simulink model "t_type_three_phase_q1q4_switching"  (R2025b)
settings: Solver=ode23t  StartTime=0.0  StopTime=0.06  MaxStep=max_step_sw  RelTol=1e-3
PreLoadFcn:
  | demo_root=fileparts(fileparts(get_param(bdroot,'FileName'))); run(fullfile(demo_root,'parameters','closed_loop_demo_parameters.m')); clear demo_root;
undefined symbols (not defined in the file): dead_time_cl, m_index, Rd_sw, T_switch, Vdc_sw, w_grid_sw
libraries: ee_lib x29, nesl_utility x19, fl_lib x7, simulink x3
settings Model: Creator=bob  LastModifiedBy=bob

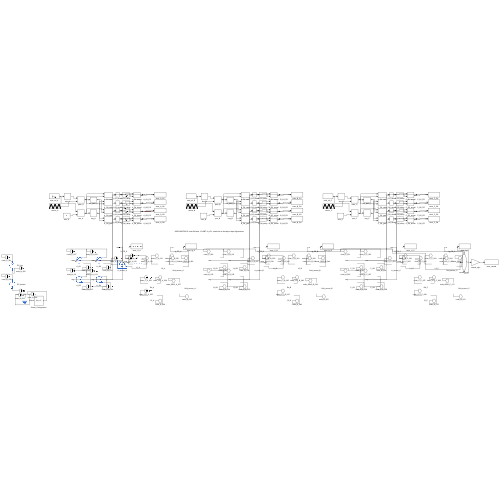
[thumbnail: Simulink's stored preview of the top-level diagram]
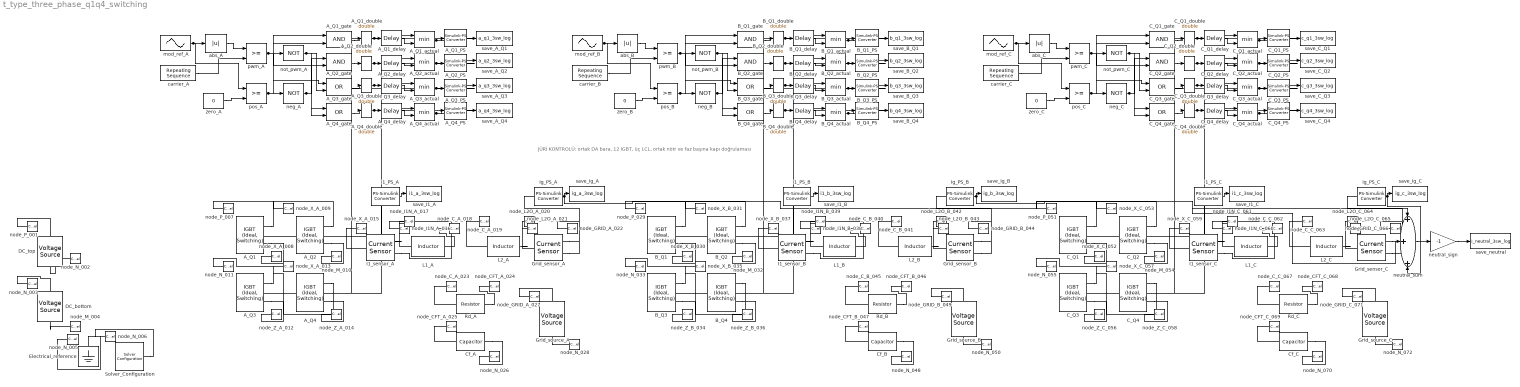
== system t_type_three_phase_q1q4_switching ==
  note: JÜRİ KONTROLÜ: ortak DA bara, 12 IGBT, üç LCL, ortak nötr ve faz başına kapı doğrulaması
  A_Q{1..4} (4 alike) : ee_lib/Semiconductors & Converters/IGBT (Ideal, Switching)  port_option=ee.enum.controlport.ps  Vf=Vf_sw V  Ron=Ron_sw Ohm  Goff=Goff_sw 1/Ohm  Vth=Vth_sw V  diode_param=ee.enum.semiconductors.protectionDiode.nodynamics  diode_Vf=0.8 V  diode_Ron=0.001 Ohm  diode_Goff=1e-5 1/Ohm  diode_C=50e-9 F  diode_iRM=-235 A  diode_iF=300 A  diode_idot=-50 A/us  diode_trr_param=ee.enum.converters.diodeReverseParam.trr_factor  diode_trr_factor=3  diode_trr=15 us  diode_Qrr=1500 s*uA  ice_specify=off  ice_priority=None  ice=0 A  ice_nominal_specify=off  ice_nominal_value=1  ice_nominal_unit=A  vce_specify=off  vce_priority=None  vce=0 V  vce_nominal_specify=off  vce_nominal_value=1  vce_nominal_unit=V  vge_specify=off  vge_priority=None  vge=0 V  vge_nominal_specify=off  vge_nominal_value=1  vge_nominal_unit=V  thermal_loss_option=ee.enum.converters.thermalLossOption.constantvalues  Von_data=[0, .1, .6, .8, 1, 1.3, 1.6, 2, 2.4; 0, .1, .7, 1, 1.2, 1.5, 1.9, 2.4, 2.8] V  Tj=[298.15, 398.15] K  Iout_data=[0, .1, 1, 5, 10, 20, 40, 70, 100] A  Eon_data=[0, .0024, .024, .12, .2, .48, 1.04, 2.16, 3.24; 0, .003, .03, .15, .25, .6, 1.3, 2.7, 4.05] * 1e-3 J  Eoff_data=[0, .0007, .0066, .033, .066, .17, .33, .83, 1.5; 0, .001, .01, .05, .1, .25, .5, 1.2, 2.2] * 1e-3 J  Eon_data_3D=[zeros(2, 9, 3)] J  Eoff_data_3D=[zeros(2, 9, 3)] J  Tj_loss=[298.15, 398.15] K  Iout_data_loss=[0, .1, 1, 5, 10, 20, 40, 70, 100] A  tabulateWithVce=false  Vce_loss=[0, 150, 300] V  Eon_scalar=22.86e-3 J  Eoff_scalar=17.14e-3 J  Voff=300 V  Iout_scalar=600 A  useCurrentFromPreviousCycle=false  useVoltageFromPreviousCycle=false  diodeModelType=ee.enum.converters.diodeModelType.pwl  diodeTableType=ee.enum.diode.tableType.IfMat  diode_ReverseIVType=ee.enum.diode.diodeReverseIV.constant  diode_IfMat=[.07, .12, .19, 1.75, 4.24, 7.32, 11.2; .16, .3, .72, 2.14, 4.02, 6.35, 9.12] A  diode_VfMat=[.9, 1.15, 1.25, 1.5, 1.75, 2.17, 2.6, 2.85; .58, .68, .75, 1.1, 1.38, 1.77, 2.27, 2.7] V  diode_TjVec=[25, 125] degC  diode_VfVec=[.5, .7, .9, 1.3, 1.7, 2.1, 2.5] V  diode_IfVec=[.1, .2, .5, 1, 2, 4, 7, 10] A  diode_IrMat=[1e-06, 2e-06, 5e-06, 1e-05, 2.5e-05, 5e-05, .0001; 2e-06, 5e-06, 1e-05, 4e-05, 8e-05, .0002, .0005] A  diode_VrMat=[10, 100, 200, 250, 300, 325, 350; 10, 70, 160, 220, 270, 300, 320] V  diode_VrVec=[10, 20, 40, 50, 70, 80, 100] V  diode_IrVec=[1e-06, 2e-06, 5e-06, 1e-05, 2e-05, 5e-05, .0001] A  diode_Vr=-600 V  diode_Ls=150 nH  diode_Erec=0.03 J  diode_rec_loss_model=ee.enum.diode.reverseRecoveryModel.fixed  diode_ErecVal=0 J  diode_scaleWithIandV=true  diode_ErecMat=zeros(2, 3) J  diode_TjrecVec=[298.15, 398.15] K  diode_IfrecVec=[.1, 1, 10] A  diode_IrecVal=10 A  diode_VrecVal=10 V  diode_tFilter=1 / 1000 / 100 s  separateThermalPortForDiode=false  thermal_network_parameterization=ee.enum.thermalNetworkTopology.external  Rth=[.08, .5] K/W  Rth_Cauer=[.08, .1, .5] K/W  Rth_Foster=[.08, .14, .22, .16] K/W  thermal_mass_parameterization=ee.enum.thermalNetwork.timeconstant  thermal_mass=[.01, .5] J/K  thermal_mass_Cauer=[.01, .1, .5] J/K  thermal_mass_Foster=[.001, .005, .05, .5] J/K  thermal_time_constant=[.001, .2] s  thermal_time_constant_Cauer=[.001, .1, .2] s  thermal_time_constant_Foster=[7e-05, .0007, .01, .08] s  thermal_mass_initial_temperatures=[25, 25] degC  thermal_mass_initial_temperatures_Cauer=[25, 25, 25] degC  junction_thermal_mass=0.01 J/K  Tvec_initial_Foster=[25, 25, 25, 25] degC  RthDiode=[.03, .2] K/W  RthCauerDiode=[.03, .1, .2] K/W  RthFosterDiode=[.03, .2] K/W  thermalMassDiode=[3, 25] J/K  thermalMassCauerDiode=[3, 10, 25] J/K  thermalMassFosterDiode=[33, 50] J/K  thermalTauDiode=[.1, 5] s  thermalTauCauerDiode=[.1, 1, 5] s  thermalTauFosterDiode=[1, 10] s  thermalMassInitTempDiode=[25, 25] degC  thermalMassInitTempCauerDiode=[25, 25, 25] degC  junctionthermalMassDiode=0.1 J/K  TVecInitialFosterDiode=[25, 25, 25, 25] degC  no_thermal_network=0  IGBT_junction_temperature_specify=off  IGBT_junction_temperature_priority=None  IGBT_junction_temperature=25 degC  IGBT_junction_temperature_nominal_specify=off  IGBT_junction_temperature_nominal_value=1  IGBT_junction_temperature_nominal_unit=degC  diode_junction_temperature_specify=off  diode_junction_temperature_priority=None  diode_junction_temperature=25 degC  diode_junction_temperature_nominal_specify=off  diode_junction_temperature_nominal_value=1  diode_junction_temperature_nominal_unit=degC  Qj_specify=off  Qj_priority=None  Qj=0 W  Qj_nominal_specify=off  Qj_nominal_value=1  Qj_nominal_unit=W  accumulatedSwitchingLosses_specify=off  accumulatedSwitchingLosses_priority=None  accumulatedSwitchingLosses=0 J
  A_Q1_PS : nesl_utility/Simulink-PS Converter  PhysicalDomain=network_engine_domain  SubClassName=ps_input  LeftPortType=input  RightPortType=output  PseudoPeriodic=off  Frequencies=[]  NoiseDistribution=none  NoiseParameters=[]  Unit=V  AffineConversion=off  FilteringAndDerivatives=zero  SimscapeFilterOrder=1  InputFilterTimeConstant=0.001  UdotUserProvided=0
  A_Q1_actual : MinMax  Inputs=2
  A_Q1_delay : TransportDelay  DelayTime=dead_time_cl
  A_Q1_double : DataTypeConversion  OutDataTypeStr=double  SaturateOnIntegerOverflow=off  RndMeth=Floor
  A_Q1_gate : Logic  AllPortsSameDT=off  OutDataTypeStr=boolean
  A_Q2_PS : nesl_utility/Simulink-PS Converter  PhysicalDomain=network_engine_domain  SubClassName=ps_input  LeftPortType=input  RightPortType=output  PseudoPeriodic=off  Frequencies=[]  NoiseDistribution=none  NoiseParameters=[]  Unit=V  AffineConversion=off  FilteringAndDerivatives=zero  SimscapeFilterOrder=1  InputFilterTimeConstant=0.001  UdotUserProvided=0
  A_Q2_actual : MinMax  Inputs=2
  A_Q2_delay : TransportDelay  DelayTime=dead_time_cl
  A_Q2_double : DataTypeConversion  OutDataTypeStr=double  SaturateOnIntegerOverflow=off  RndMeth=Floor
  A_Q2_gate : Logic  AllPortsSameDT=off  OutDataTypeStr=boolean
  A_Q3_PS : nesl_utility/Simulink-PS Converter  PhysicalDomain=network_engine_domain  SubClassName=ps_input  LeftPortType=input  RightPortType=output  PseudoPeriodic=off  Frequencies=[]  NoiseDistribution=none  NoiseParameters=[]  Unit=V  AffineConversion=off  FilteringAndDerivatives=zero  SimscapeFilterOrder=1  InputFilterTimeConstant=0.001  UdotUserProvided=0
  A_Q3_actual : MinMax  Inputs=2
  A_Q3_delay : TransportDelay  DelayTime=dead_time_cl
  A_Q3_double : DataTypeConversion  OutDataTypeStr=double  SaturateOnIntegerOverflow=off  RndMeth=Floor
  A_Q3_gate : Logic  Operator=OR  AllPortsSameDT=off  OutDataTypeStr=boolean
  A_Q4_PS : nesl_utility/Simulink-PS Converter  PhysicalDomain=network_engine_domain  SubClassName=ps_input  LeftPortType=input  RightPortType=output  PseudoPeriodic=off  Frequencies=[]  NoiseDistribution=none  NoiseParameters=[]  Unit=V  AffineConversion=off  FilteringAndDerivatives=zero  SimscapeFilterOrder=1  InputFilterTimeConstant=0.001  UdotUserProvided=0
  A_Q4_actual : MinMax  Inputs=2
  A_Q4_delay : TransportDelay  DelayTime=dead_time_cl
  A_Q4_double : DataTypeConversion  OutDataTypeStr=double  SaturateOnIntegerOverflow=off  RndMeth=Floor
  A_Q4_gate : Logic  Operator=OR  AllPortsSameDT=off  OutDataTypeStr=boolean
  B_Q{1..4} (4 alike) : ee_lib/Semiconductors & Converters/IGBT (Ideal, Switching)  port_option=ee.enum.controlport.ps  Vf=Vf_sw V  Ron=Ron_sw Ohm  Goff=Goff_sw 1/Ohm  Vth=Vth_sw V  diode_param=ee.enum.semiconductors.protectionDiode.nodynamics  diode_Vf=0.8 V  diode_Ron=0.001 Ohm  diode_Goff=1e-5 1/Ohm  diode_C=50e-9 F  diode_iRM=-235 A  diode_iF=300 A  diode_idot=-50 A/us  diode_trr_param=ee.enum.converters.diodeReverseParam.trr_factor  diode_trr_factor=3  diode_trr=15 us  diode_Qrr=1500 s*uA  ice_specify=off  ice_priority=None  ice=0 A  ice_nominal_specify=off  ice_nominal_value=1  ice_nominal_unit=A  vce_specify=off  vce_priority=None  vce=0 V  vce_nominal_specify=off  vce_nominal_value=1  vce_nominal_unit=V  vge_specify=off  vge_priority=None  vge=0 V  vge_nominal_specify=off  vge_nominal_value=1  vge_nominal_unit=V  thermal_loss_option=ee.enum.converters.thermalLossOption.constantvalues  Von_data=[0, .1, .6, .8, 1, 1.3, 1.6, 2, 2.4; 0, .1, .7, 1, 1.2, 1.5, 1.9, 2.4, 2.8] V  Tj=[298.15, 398.15] K  Iout_data=[0, .1, 1, 5, 10, 20, 40, 70, 100] A  Eon_data=[0, .0024, .024, .12, .2, .48, 1.04, 2.16, 3.24; 0, .003, .03, .15, .25, .6, 1.3, 2.7, 4.05] * 1e-3 J  Eoff_data=[0, .0007, .0066, .033, .066, .17, .33, .83, 1.5; 0, .001, .01, .05, .1, .25, .5, 1.2, 2.2] * 1e-3 J  Eon_data_3D=[zeros(2, 9, 3)] J  Eoff_data_3D=[zeros(2, 9, 3)] J  Tj_loss=[298.15, 398.15] K  Iout_data_loss=[0, .1, 1, 5, 10, 20, 40, 70, 100] A  tabulateWithVce=false  Vce_loss=[0, 150, 300] V  Eon_scalar=22.86e-3 J  Eoff_scalar=17.14e-3 J  Voff=300 V  Iout_scalar=600 A  useCurrentFromPreviousCycle=false  useVoltageFromPreviousCycle=false  diodeModelType=ee.enum.converters.diodeModelType.pwl  diodeTableType=ee.enum.diode.tableType.IfMat  diode_ReverseIVType=ee.enum.diode.diodeReverseIV.constant  diode_IfMat=[.07, .12, .19, 1.75, 4.24, 7.32, 11.2; .16, .3, .72, 2.14, 4.02, 6.35, 9.12] A  diode_VfMat=[.9, 1.15, 1.25, 1.5, 1.75, 2.17, 2.6, 2.85; .58, .68, .75, 1.1, 1.38, 1.77, 2.27, 2.7] V  diode_TjVec=[25, 125] degC  diode_VfVec=[.5, .7, .9, 1.3, 1.7, 2.1, 2.5] V  diode_IfVec=[.1, .2, .5, 1, 2, 4, 7, 10] A  diode_IrMat=[1e-06, 2e-06, 5e-06, 1e-05, 2.5e-05, 5e-05, .0001; 2e-06, 5e-06, 1e-05, 4e-05, 8e-05, .0002, .0005] A  diode_VrMat=[10, 100, 200, 250, 300, 325, 350; 10, 70, 160, 220, 270, 300, 320] V  diode_VrVec=[10, 20, 40, 50, 70, 80, 100] V  diode_IrVec=[1e-06, 2e-06, 5e-06, 1e-05, 2e-05, 5e-05, .0001] A  diode_Vr=-600 V  diode_Ls=150 nH  diode_Erec=0.03 J  diode_rec_loss_model=ee.enum.diode.reverseRecoveryModel.fixed  diode_ErecVal=0 J  diode_scaleWithIandV=true  diode_ErecMat=zeros(2, 3) J  diode_TjrecVec=[298.15, 398.15] K  diode_IfrecVec=[.1, 1, 10] A  diode_IrecVal=10 A  diode_VrecVal=10 V  diode_tFilter=1 / 1000 / 100 s  separateThermalPortForDiode=false  thermal_network_parameterization=ee.enum.thermalNetworkTopology.external  Rth=[.08, .5] K/W  Rth_Cauer=[.08, .1, .5] K/W  Rth_Foster=[.08, .14, .22, .16] K/W  thermal_mass_parameterization=ee.enum.thermalNetwork.timeconstant  thermal_mass=[.01, .5] J/K  thermal_mass_Cauer=[.01, .1, .5] J/K  thermal_mass_Foster=[.001, .005, .05, .5] J/K  thermal_time_constant=[.001, .2] s  thermal_time_constant_Cauer=[.001, .1, .2] s  thermal_time_constant_Foster=[7e-05, .0007, .01, .08] s  thermal_mass_initial_temperatures=[25, 25] degC  thermal_mass_initial_temperatures_Cauer=[25, 25, 25] degC  junction_thermal_mass=0.01 J/K  Tvec_initial_Foster=[25, 25, 25, 25] degC  RthDiode=[.03, .2] K/W  RthCauerDiode=[.03, .1, .2] K/W  RthFosterDiode=[.03, .2] K/W  thermalMassDiode=[3, 25] J/K  thermalMassCauerDiode=[3, 10, 25] J/K  thermalMassFosterDiode=[33, 50] J/K  thermalTauDiode=[.1, 5] s  thermalTauCauerDiode=[.1, 1, 5] s  thermalTauFosterDiode=[1, 10] s  thermalMassInitTempDiode=[25, 25] degC  thermalMassInitTempCauerDiode=[25, 25, 25] degC  junctionthermalMassDiode=0.1 J/K  TVecInitialFosterDiode=[25, 25, 25, 25] degC  no_thermal_network=0  IGBT_junction_temperature_specify=off  IGBT_junction_temperature_priority=None  IGBT_junction_temperature=25 degC  IGBT_junction_temperature_nominal_specify=off  IGBT_junction_temperature_nominal_value=1  IGBT_junction_temperature_nominal_unit=degC  diode_junction_temperature_specify=off  diode_junction_temperature_priority=None  diode_junction_temperature=25 degC  diode_junction_temperature_nominal_specify=off  diode_junction_temperature_nominal_value=1  diode_junction_temperature_nominal_unit=degC  Qj_specify=off  Qj_priority=None  Qj=0 W  Qj_nominal_specify=off  Qj_nominal_value=1  Qj_nominal_unit=W  accumulatedSwitchingLosses_specify=off  accumulatedSwitchingLosses_priority=None  accumulatedSwitchingLosses=0 J
  B_Q1_PS : nesl_utility/Simulink-PS Converter  PhysicalDomain=network_engine_domain  SubClassName=ps_input  LeftPortType=input  RightPortType=output  PseudoPeriodic=off  Frequencies=[]  NoiseDistribution=none  NoiseParameters=[]  Unit=V  AffineConversion=off  FilteringAndDerivatives=zero  SimscapeFilterOrder=1  InputFilterTimeConstant=0.001  UdotUserProvided=0
  B_Q1_actual : MinMax  Inputs=2
  B_Q1_delay : TransportDelay  DelayTime=dead_time_cl
  B_Q1_double : DataTypeConversion  OutDataTypeStr=double  SaturateOnIntegerOverflow=off  RndMeth=Floor
  B_Q1_gate : Logic  AllPortsSameDT=off  OutDataTypeStr=boolean
  B_Q2_PS : nesl_utility/Simulink-PS Converter  PhysicalDomain=network_engine_domain  SubClassName=ps_input  LeftPortType=input  RightPortType=output  PseudoPeriodic=off  Frequencies=[]  NoiseDistribution=none  NoiseParameters=[]  Unit=V  AffineConversion=off  FilteringAndDerivatives=zero  SimscapeFilterOrder=1  InputFilterTimeConstant=0.001  UdotUserProvided=0
  B_Q2_actual : MinMax  Inputs=2
  B_Q2_delay : TransportDelay  DelayTime=dead_time_cl
  B_Q2_double : DataTypeConversion  OutDataTypeStr=double  SaturateOnIntegerOverflow=off  RndMeth=Floor
  B_Q2_gate : Logic  AllPortsSameDT=off  OutDataTypeStr=boolean
  B_Q3_PS : nesl_utility/Simulink-PS Converter  PhysicalDomain=network_engine_domain  SubClassName=ps_input  LeftPortType=input  RightPortType=output  PseudoPeriodic=off  Frequencies=[]  NoiseDistribution=none  NoiseParameters=[]  Unit=V  AffineConversion=off  FilteringAndDerivatives=zero  SimscapeFilterOrder=1  InputFilterTimeConstant=0.001  UdotUserProvided=0
  B_Q3_actual : MinMax  Inputs=2
  B_Q3_delay : TransportDelay  DelayTime=dead_time_cl
  B_Q3_double : DataTypeConversion  OutDataTypeStr=double  SaturateOnIntegerOverflow=off  RndMeth=Floor
  B_Q3_gate : Logic  Operator=OR  AllPortsSameDT=off  OutDataTypeStr=boolean
  B_Q4_PS : nesl_utility/Simulink-PS Converter  PhysicalDomain=network_engine_domain  SubClassName=ps_input  LeftPortType=input  RightPortType=output  PseudoPeriodic=off  Frequencies=[]  NoiseDistribution=none  NoiseParameters=[]  Unit=V  AffineConversion=off  FilteringAndDerivatives=zero  SimscapeFilterOrder=1  InputFilterTimeConstant=0.001  UdotUserProvided=0
  B_Q4_actual : MinMax  Inputs=2
  B_Q4_delay : TransportDelay  DelayTime=dead_time_cl
  B_Q4_double : DataTypeConversion  OutDataTypeStr=double  SaturateOnIntegerOverflow=off  RndMeth=Floor
  B_Q4_gate : Logic  Operator=OR  AllPortsSameDT=off  OutDataTypeStr=boolean
  C_Q{1..4} (4 alike) : ee_lib/Semiconductors & Converters/IGBT (Ideal, Switching)  port_option=ee.enum.controlport.ps  Vf=Vf_sw V  Ron=Ron_sw Ohm  Goff=Goff_sw 1/Ohm  Vth=Vth_sw V  diode_param=ee.enum.semiconductors.protectionDiode.nodynamics  diode_Vf=0.8 V  diode_Ron=0.001 Ohm  diode_Goff=1e-5 1/Ohm  diode_C=50e-9 F  diode_iRM=-235 A  diode_iF=300 A  diode_idot=-50 A/us  diode_trr_param=ee.enum.converters.diodeReverseParam.trr_factor  diode_trr_factor=3  diode_trr=15 us  diode_Qrr=1500 s*uA  ice_specify=off  ice_priority=None  ice=0 A  ice_nominal_specify=off  ice_nominal_value=1  ice_nominal_unit=A  vce_specify=off  vce_priority=None  vce=0 V  vce_nominal_specify=off  vce_nominal_value=1  vce_nominal_unit=V  vge_specify=off  vge_priority=None  vge=0 V  vge_nominal_specify=off  vge_nominal_value=1  vge_nominal_unit=V  thermal_loss_option=ee.enum.converters.thermalLossOption.constantvalues  Von_data=[0, .1, .6, .8, 1, 1.3, 1.6, 2, 2.4; 0, .1, .7, 1, 1.2, 1.5, 1.9, 2.4, 2.8] V  Tj=[298.15, 398.15] K  Iout_data=[0, .1, 1, 5, 10, 20, 40, 70, 100] A  Eon_data=[0, .0024, .024, .12, .2, .48, 1.04, 2.16, 3.24; 0, .003, .03, .15, .25, .6, 1.3, 2.7, 4.05] * 1e-3 J  Eoff_data=[0, .0007, .0066, .033, .066, .17, .33, .83, 1.5; 0, .001, .01, .05, .1, .25, .5, 1.2, 2.2] * 1e-3 J  Eon_data_3D=[zeros(2, 9, 3)] J  Eoff_data_3D=[zeros(2, 9, 3)] J  Tj_loss=[298.15, 398.15] K  Iout_data_loss=[0, .1, 1, 5, 10, 20, 40, 70, 100] A  tabulateWithVce=false  Vce_loss=[0, 150, 300] V  Eon_scalar=22.86e-3 J  Eoff_scalar=17.14e-3 J  Voff=300 V  Iout_scalar=600 A  useCurrentFromPreviousCycle=false  useVoltageFromPreviousCycle=false  diodeModelType=ee.enum.converters.diodeModelType.pwl  diodeTableType=ee.enum.diode.tableType.IfMat  diode_ReverseIVType=ee.enum.diode.diodeReverseIV.constant  diode_IfMat=[.07, .12, .19, 1.75, 4.24, 7.32, 11.2; .16, .3, .72, 2.14, 4.02, 6.35, 9.12] A  diode_VfMat=[.9, 1.15, 1.25, 1.5, 1.75, 2.17, 2.6, 2.85; .58, .68, .75, 1.1, 1.38, 1.77, 2.27, 2.7] V  diode_TjVec=[25, 125] degC  diode_VfVec=[.5, .7, .9, 1.3, 1.7, 2.1, 2.5] V  diode_IfVec=[.1, .2, .5, 1, 2, 4, 7, 10] A  diode_IrMat=[1e-06, 2e-06, 5e-06, 1e-05, 2.5e-05, 5e-05, .0001; 2e-06, 5e-06, 1e-05, 4e-05, 8e-05, .0002, .0005] A  diode_VrMat=[10, 100, 200, 250, 300, 325, 350; 10, 70, 160, 220, 270, 300, 320] V  diode_VrVec=[10, 20, 40, 50, 70, 80, 100] V  diode_IrVec=[1e-06, 2e-06, 5e-06, 1e-05, 2e-05, 5e-05, .0001] A  diode_Vr=-600 V  diode_Ls=150 nH  diode_Erec=0.03 J  diode_rec_loss_model=ee.enum.diode.reverseRecoveryModel.fixed  diode_ErecVal=0 J  diode_scaleWithIandV=true  diode_ErecMat=zeros(2, 3) J  diode_TjrecVec=[298.15, 398.15] K  diode_IfrecVec=[.1, 1, 10] A  diode_IrecVal=10 A  diode_VrecVal=10 V  diode_tFilter=1 / 1000 / 100 s  separateThermalPortForDiode=false  thermal_network_parameterization=ee.enum.thermalNetworkTopology.external  Rth=[.08, .5] K/W  Rth_Cauer=[.08, .1, .5] K/W  Rth_Foster=[.08, .14, .22, .16] K/W  thermal_mass_parameterization=ee.enum.thermalNetwork.timeconstant  thermal_mass=[.01, .5] J/K  thermal_mass_Cauer=[.01, .1, .5] J/K  thermal_mass_Foster=[.001, .005, .05, .5] J/K  thermal_time_constant=[.001, .2] s  thermal_time_constant_Cauer=[.001, .1, .2] s  thermal_time_constant_Foster=[7e-05, .0007, .01, .08] s  thermal_mass_initial_temperatures=[25, 25] degC  thermal_mass_initial_temperatures_Cauer=[25, 25, 25] degC  junction_thermal_mass=0.01 J/K  Tvec_initial_Foster=[25, 25, 25, 25] degC  RthDiode=[.03, .2] K/W  RthCauerDiode=[.03, .1, .2] K/W  RthFosterDiode=[.03, .2] K/W  thermalMassDiode=[3, 25] J/K  thermalMassCauerDiode=[3, 10, 25] J/K  thermalMassFosterDiode=[33, 50] J/K  thermalTauDiode=[.1, 5] s  thermalTauCauerDiode=[.1, 1, 5] s  thermalTauFosterDiode=[1, 10] s  thermalMassInitTempDiode=[25, 25] degC  thermalMassInitTempCauerDiode=[25, 25, 25] degC  junctionthermalMassDiode=0.1 J/K  TVecInitialFosterDiode=[25, 25, 25, 25] degC  no_thermal_network=0  IGBT_junction_temperature_specify=off  IGBT_junction_temperature_priority=None  IGBT_junction_temperature=25 degC  IGBT_junction_temperature_nominal_specify=off  IGBT_junction_temperature_nominal_value=1  IGBT_junction_temperature_nominal_unit=degC  diode_junction_temperature_specify=off  diode_junction_temperature_priority=None  diode_junction_temperature=25 degC  diode_junction_temperature_nominal_specify=off  diode_junction_temperature_nominal_value=1  diode_junction_temperature_nominal_unit=degC  Qj_specify=off  Qj_priority=None  Qj=0 W  Qj_nominal_specify=off  Qj_nominal_value=1  Qj_nominal_unit=W  accumulatedSwitchingLosses_specify=off  accumulatedSwitchingLosses_priority=None  accumulatedSwitchingLosses=0 J
  C_Q1_PS : nesl_utility/Simulink-PS Converter  PhysicalDomain=network_engine_domain  SubClassName=ps_input  LeftPortType=input  RightPortType=output  PseudoPeriodic=off  Frequencies=[]  NoiseDistribution=none  NoiseParameters=[]  Unit=V  AffineConversion=off  FilteringAndDerivatives=zero  SimscapeFilterOrder=1  InputFilterTimeConstant=0.001  UdotUserProvided=0
  C_Q1_actual : MinMax  Inputs=2
  C_Q1_delay : TransportDelay  DelayTime=dead_time_cl
  C_Q1_double : DataTypeConversion  OutDataTypeStr=double  SaturateOnIntegerOverflow=off  RndMeth=Floor
  C_Q1_gate : Logic  AllPortsSameDT=off  OutDataTypeStr=boolean
  C_Q2_PS : nesl_utility/Simulink-PS Converter  PhysicalDomain=network_engine_domain  SubClassName=ps_input  LeftPortType=input  RightPortType=output  PseudoPeriodic=off  Frequencies=[]  NoiseDistribution=none  NoiseParameters=[]  Unit=V  AffineConversion=off  FilteringAndDerivatives=zero  SimscapeFilterOrder=1  InputFilterTimeConstant=0.001  UdotUserProvided=0
  C_Q2_actual : MinMax  Inputs=2
  C_Q2_delay : TransportDelay  DelayTime=dead_time_cl
  C_Q2_double : DataTypeConversion  OutDataTypeStr=double  SaturateOnIntegerOverflow=off  RndMeth=Floor
  C_Q2_gate : Logic  AllPortsSameDT=off  OutDataTypeStr=boolean
  C_Q3_PS : nesl_utility/Simulink-PS Converter  PhysicalDomain=network_engine_domain  SubClassName=ps_input  LeftPortType=input  RightPortType=output  PseudoPeriodic=off  Frequencies=[]  NoiseDistribution=none  NoiseParameters=[]  Unit=V  AffineConversion=off  FilteringAndDerivatives=zero  SimscapeFilterOrder=1  InputFilterTimeConstant=0.001  UdotUserProvided=0
  C_Q3_actual : MinMax  Inputs=2
  C_Q3_delay : TransportDelay  DelayTime=dead_time_cl
  C_Q3_double : DataTypeConversion  OutDataTypeStr=double  SaturateOnIntegerOverflow=off  RndMeth=Floor
  C_Q3_gate : Logic  Operator=OR  AllPortsSameDT=off  OutDataTypeStr=boolean
  C_Q4_PS : nesl_utility/Simulink-PS Converter  PhysicalDomain=network_engine_domain  SubClassName=ps_input  LeftPortType=input  RightPortType=output  PseudoPeriodic=off  Frequencies=[]  NoiseDistribution=none  NoiseParameters=[]  Unit=V  AffineConversion=off  FilteringAndDerivatives=zero  SimscapeFilterOrder=1  InputFilterTimeConstant=0.001  UdotUserProvided=0
  C_Q4_actual : MinMax  Inputs=2
  C_Q4_delay : TransportDelay  DelayTime=dead_time_cl
  C_Q4_double : DataTypeConversion  OutDataTypeStr=double  SaturateOnIntegerOverflow=off  RndMeth=Floor
  C_Q4_gate : Logic  Operator=OR  AllPortsSameDT=off  OutDataTypeStr=boolean
  Cf_A : ee_lib/Passive/Capacitor  cap_option=ee.enum.passive.capacitor.capOption.const  c=Cf_sw F  Cvec=[1e-05, 1e-06] F  Vvec=[0, 10] V  CV_table_symmetry=ee.enum.passive.capacitor.tableSymmetry.yes  f_vec=[1, 10] kHz  DFext_vec=[.8, 1.2]  enable_C_tol=ee.enum.toleranceApplication.none  averaging_period=0 s  C_tol=5  tol_distribution=ee.enum.toleranceDistribution.uniform  nSigma=4  r=0 Ohm  g=0 1/Ohm  enable_operating_limits=ee.enum.enable.no  operating_limit_action=ee.enum.passive.reportOpLim.warn  max_working_voltage_range=[-25, 25] V  power_rating=1 W  maxTemperature=85 degC  thermalEnable=false  thermalMass=1 J/K  i_specify=off  i_priority=None  i=0 A  i_nominal_specify=off  i_nominal_value=1  i_nominal_unit=A  v_specify=off  v_priority=None  v=0 V  v_nominal_specify=off  v_nominal_value=1  v_nominal_unit=V  vc_specify=off  vc_priority=High  vc=0 V  vc_nominal_specify=off  vc_nominal_value=1  vc_nominal_unit=V  T_specify=off  T_priority=None  T=298.15 K  T_nominal_specify=off  T_nominal_value=1  T_nominal_unit=K
  Cf_B : ee_lib/Passive/Capacitor  cap_option=ee.enum.passive.capacitor.capOption.const  c=Cf_sw F  Cvec=[1e-05, 1e-06] F  Vvec=[0, 10] V  CV_table_symmetry=ee.enum.passive.capacitor.tableSymmetry.yes  f_vec=[1, 10] kHz  DFext_vec=[.8, 1.2]  enable_C_tol=ee.enum.toleranceApplication.none  averaging_period=0 s  C_tol=5  tol_distribution=ee.enum.toleranceDistribution.uniform  nSigma=4  r=0 Ohm  g=0 1/Ohm  enable_operating_limits=ee.enum.enable.no  operating_limit_action=ee.enum.passive.reportOpLim.warn  max_working_voltage_range=[-25, 25] V  power_rating=1 W  maxTemperature=85 degC  thermalEnable=false  thermalMass=1 J/K  i_specify=off  i_priority=None  i=0 A  i_nominal_specify=off  i_nominal_value=1  i_nominal_unit=A  v_specify=off  v_priority=None  v=0 V  v_nominal_specify=off  v_nominal_value=1  v_nominal_unit=V  vc_specify=off  vc_priority=High  vc=0 V  vc_nominal_specify=off  vc_nominal_value=1  vc_nominal_unit=V  T_specify=off  T_priority=None  T=298.15 K  T_nominal_specify=off  T_nominal_value=1  T_nominal_unit=K
  Cf_C : ee_lib/Passive/Capacitor  cap_option=ee.enum.passive.capacitor.capOption.const  c=Cf_sw F  Cvec=[1e-05, 1e-06] F  Vvec=[0, 10] V  CV_table_symmetry=ee.enum.passive.capacitor.tableSymmetry.yes  f_vec=[1, 10] kHz  DFext_vec=[.8, 1.2]  enable_C_tol=ee.enum.toleranceApplication.none  averaging_period=0 s  C_tol=5  tol_distribution=ee.enum.toleranceDistribution.uniform  nSigma=4  r=0 Ohm  g=0 1/Ohm  enable_operating_limits=ee.enum.enable.no  operating_limit_action=ee.enum.passive.reportOpLim.warn  max_working_voltage_range=[-25, 25] V  power_rating=1 W  maxTemperature=85 degC  thermalEnable=false  thermalMass=1 J/K  i_specify=off  i_priority=None  i=0 A  i_nominal_specify=off  i_nominal_value=1  i_nominal_unit=A  v_specify=off  v_priority=None  v=0 V  v_nominal_specify=off  v_nominal_value=1  v_nominal_unit=V  vc_specify=off  vc_priority=High  vc=0 V  vc_nominal_specify=off  vc_nominal_value=1  vc_nominal_unit=V  T_specify=off  T_priority=None  T=298.15 K  T_nominal_specify=off  T_nominal_value=1  T_nominal_unit=K
  DC_bottom : ee_lib/Sources/Voltage Source  dc_voltage=Vdc_sw/2 V  ac_voltage=0 V  ac_shift=0 rad  ac_frequency=60 Hz  noise_mode=ee.enum.sources.noise.Disabled  PSD=0 V^2/Hz  sample_time=1e-3 s  repeatability=ee.enum.sources.repeatability.NotRepeatable  user_seed=0  auto_seed=3890346746  i_specify=off  i_priority=None  i=0 A  i_nominal_specify=off  i_nominal_value=1  i_nominal_unit=A  v_specify=off  v_priority=None  v=0 V  v_nominal_specify=off  v_nominal_value=1  v_nominal_unit=V
  DC_top : ee_lib/Sources/Voltage Source  dc_voltage=Vdc_sw/2 V  ac_voltage=0 V  ac_shift=0 rad  ac_frequency=60 Hz  noise_mode=ee.enum.sources.noise.Disabled  PSD=0 V^2/Hz  sample_time=1e-3 s  repeatability=ee.enum.sources.repeatability.NotRepeatable  user_seed=0  auto_seed=3499211588  i_specify=off  i_priority=None  i=0 A  i_nominal_specify=off  i_nominal_value=1  i_nominal_unit=A  v_specify=off  v_priority=None  v=0 V  v_nominal_specify=off  v_nominal_value=1  v_nominal_unit=V
  Electrical_reference : fl_lib/Electrical/Electrical Elements/Electrical Reference
  Grid_sensor_A : fl_lib/Electrical/Electrical Sensors/Current Sensor
  Grid_sensor_B : fl_lib/Electrical/Electrical Sensors/Current Sensor
  Grid_sensor_C : fl_lib/Electrical/Electrical Sensors/Current Sensor
  Grid_source_A : ee_lib/Sources/Voltage Source  dc_voltage=0 V  ac_voltage=V_grid_pk_sw V  ac_shift=0 rad  ac_frequency=f_grid_sw Hz  noise_mode=ee.enum.sources.noise.Disabled  PSD=0 V^2/Hz  sample_time=1e-3 s  repeatability=ee.enum.sources.repeatability.NotRepeatable  user_seed=0  auto_seed=3922919431  i_specify=off  i_priority=None  i=0 A  i_nominal_specify=off  i_nominal_value=1  i_nominal_unit=A  v_specify=off  v_priority=None  v=0 V  v_nominal_specify=off  v_nominal_value=1  v_nominal_unit=V
  Grid_source_B : ee_lib/Sources/Voltage Source  dc_voltage=0 V  ac_voltage=V_grid_pk_sw V  ac_shift=-2.0943951023931953 rad  ac_frequency=f_grid_sw Hz  noise_mode=ee.enum.sources.noise.Disabled  PSD=0 V^2/Hz  sample_time=1e-3 s  repeatability=ee.enum.sources.repeatability.NotRepeatable  user_seed=0  auto_seed=418932850  i_specify=off  i_priority=None  i=0 A  i_nominal_specify=off  i_nominal_value=1  i_nominal_unit=A  v_specify=off  v_priority=None  v=0 V  v_nominal_specify=off  v_nominal_value=1  v_nominal_unit=V
  Grid_source_C : ee_lib/Sources/Voltage Source  dc_voltage=0 V  ac_voltage=V_grid_pk_sw V  ac_shift=2.0943951023931953 rad  ac_frequency=f_grid_sw Hz  noise_mode=ee.enum.sources.noise.Disabled  PSD=0 V^2/Hz  sample_time=1e-3 s  repeatability=ee.enum.sources.repeatability.NotRepeatable  user_seed=0  auto_seed=2348838240  i_specify=off  i_priority=None  i=0 A  i_nominal_specify=off  i_nominal_value=1  i_nominal_unit=A  v_specify=off  v_priority=None  v=0 V  v_nominal_specify=off  v_nominal_value=1  v_nominal_unit=V
  I1_PS_A : nesl_utility/PS-Simulink Converter  PhysicalDomain=network_engine_domain  SubClassName=ps_output  LeftPortType=input  RightPortType=output  PseudoPeriodic=off  Frequencies=[]  VectorFormat=inherit  Unit=A  AffineConversion=off
  I1_PS_B : nesl_utility/PS-Simulink Converter  PhysicalDomain=network_engine_domain  SubClassName=ps_output  LeftPortType=input  RightPortType=output  PseudoPeriodic=off  Frequencies=[]  VectorFormat=inherit  Unit=A  AffineConversion=off
  I1_PS_C : nesl_utility/PS-Simulink Converter  PhysicalDomain=network_engine_domain  SubClassName=ps_output  LeftPortType=input  RightPortType=output  PseudoPeriodic=off  Frequencies=[]  VectorFormat=inherit  Unit=A  AffineConversion=off
  I1_sensor_A : fl_lib/Electrical/Electrical Sensors/Current Sensor
  I1_sensor_B : fl_lib/Electrical/Electrical Sensors/Current Sensor
  I1_sensor_C : fl_lib/Electrical/Electrical Sensors/Current Sensor
  Ig_PS_A : nesl_utility/PS-Simulink Converter  PhysicalDomain=network_engine_domain  SubClassName=ps_output  LeftPortType=input  RightPortType=output  PseudoPeriodic=off  Frequencies=[]  VectorFormat=inherit  Unit=A  AffineConversion=off
  Ig_PS_B : nesl_utility/PS-Simulink Converter  PhysicalDomain=network_engine_domain  SubClassName=ps_output  LeftPortType=input  RightPortType=output  PseudoPeriodic=off  Frequencies=[]  VectorFormat=inherit  Unit=A  AffineConversion=off
  Ig_PS_C : nesl_utility/PS-Simulink Converter  PhysicalDomain=network_engine_domain  SubClassName=ps_output  LeftPortType=input  RightPortType=output  PseudoPeriodic=off  Frequencies=[]  VectorFormat=inherit  Unit=A  AffineConversion=off
  L1_A : ee_lib/Passive/Inductor  l=L1_sw H  enable_L_tol=ee.enum.toleranceApplication.none  L_tol=20  tol_distribution=ee.enum.toleranceDistribution.uniform  nSigma=4  r=R1_sw Ohm  g=1e-9 1/Ohm  enable_operating_limits=ee.enum.enable.no  operating_limit_action=ee.enum.passive.reportOpLim.warn  max_working_current=1 A  power_rating=1 W  i_L_specify=off  i_L_priority=High  i_L=0 A  i_L_nominal_specify=off  i_L_nominal_value=1  i_L_nominal_unit=A
  L1_B : ee_lib/Passive/Inductor  l=L1_sw H  enable_L_tol=ee.enum.toleranceApplication.none  L_tol=20  tol_distribution=ee.enum.toleranceDistribution.uniform  nSigma=4  r=R1_sw Ohm  g=1e-9 1/Ohm  enable_operating_limits=ee.enum.enable.no  operating_limit_action=ee.enum.passive.reportOpLim.warn  max_working_current=1 A  power_rating=1 W  i_L_specify=off  i_L_priority=High  i_L=0 A  i_L_nominal_specify=off  i_L_nominal_value=1  i_L_nominal_unit=A
  L1_C : ee_lib/Passive/Inductor  l=L1_sw H  enable_L_tol=ee.enum.toleranceApplication.none  L_tol=20  tol_distribution=ee.enum.toleranceDistribution.uniform  nSigma=4  r=R1_sw Ohm  g=1e-9 1/Ohm  enable_operating_limits=ee.enum.enable.no  operating_limit_action=ee.enum.passive.reportOpLim.warn  max_working_current=1 A  power_rating=1 W  i_L_specify=off  i_L_priority=High  i_L=0 A  i_L_nominal_specify=off  i_L_nominal_value=1  i_L_nominal_unit=A
  L2_A : ee_lib/Passive/Inductor  l=L2_sw H  enable_L_tol=ee.enum.toleranceApplication.none  L_tol=20  tol_distribution=ee.enum.toleranceDistribution.uniform  nSigma=4  r=R2_sw Ohm  g=1e-9 1/Ohm  enable_operating_limits=ee.enum.enable.no  operating_limit_action=ee.enum.passive.reportOpLim.warn  max_working_current=1 A  power_rating=1 W  i_L_specify=off  i_L_priority=High  i_L=0 A  i_L_nominal_specify=off  i_L_nominal_value=1  i_L_nominal_unit=A
  L2_B : ee_lib/Passive/Inductor  l=L2_sw H  enable_L_tol=ee.enum.toleranceApplication.none  L_tol=20  tol_distribution=ee.enum.toleranceDistribution.uniform  nSigma=4  r=R2_sw Ohm  g=1e-9 1/Ohm  enable_operating_limits=ee.enum.enable.no  operating_limit_action=ee.enum.passive.reportOpLim.warn  max_working_current=1 A  power_rating=1 W  i_L_specify=off  i_L_priority=High  i_L=0 A  i_L_nominal_specify=off  i_L_nominal_value=1  i_L_nominal_unit=A
  L2_C : ee_lib/Passive/Inductor  l=L2_sw H  enable_L_tol=ee.enum.toleranceApplication.none  L_tol=20  tol_distribution=ee.enum.toleranceDistribution.uniform  nSigma=4  r=R2_sw Ohm  g=1e-9 1/Ohm  enable_operating_limits=ee.enum.enable.no  operating_limit_action=ee.enum.passive.reportOpLim.warn  max_working_current=1 A  power_rating=1 W  i_L_specify=off  i_L_priority=High  i_L=0 A  i_L_nominal_specify=off  i_L_nominal_value=1  i_L_nominal_unit=A
  Rd_A : ee_lib/Passive/Resistor  R=Rd_sw Ohm  enable_R_tol=ee.enum.toleranceApplication.none  R_tol=5  tol_distribution=ee.enum.toleranceDistribution.uniform  nSigma=4  enable_operating_limits=ee.enum.enable.no  operating_limit_action=ee.enum.passive.reportOpLim.warn  power_rating=1 W  max_working_voltage=100 V  noise_mode=ee.enum.sources.noise.Disabled  Tdevice=25 degC  sample_time=1e-3 s  repeatability=ee.enum.ic.repeatability.notRepeatable  user_seed=0  auto_seed=545404223  power_derating_T1=70 degC  power_derating_T2=155 degC  operating_temperature_range_vec=[-50, 150] degC  alpha=3.93e-3 1/K  Tmeas=25 degC  thermal_mass=100 J/K  temperature_specify=off  temperature_priority=High  temperature=298.15 K  temperature_nominal_specify=off  temperature_nominal_value=1  temperature_nominal_unit=K
  Rd_B : ee_lib/Passive/Resistor  R=Rd_sw Ohm  enable_R_tol=ee.enum.toleranceApplication.none  R_tol=5  tol_distribution=ee.enum.toleranceDistribution.uniform  nSigma=4  enable_operating_limits=ee.enum.enable.no  operating_limit_action=ee.enum.passive.reportOpLim.warn  power_rating=1 W  max_working_voltage=100 V  noise_mode=ee.enum.sources.noise.Disabled  Tdevice=25 degC  sample_time=1e-3 s  repeatability=ee.enum.ic.repeatability.notRepeatable  user_seed=0  auto_seed=2715962282  power_derating_T1=70 degC  power_derating_T2=155 degC  operating_temperature_range_vec=[-50, 150] degC  alpha=3.93e-3 1/K  Tmeas=25 degC  thermal_mass=100 J/K  temperature_specify=off  temperature_priority=High  temperature=298.15 K  temperature_nominal_specify=off  temperature_nominal_value=1  temperature_nominal_unit=K
  Rd_C : ee_lib/Passive/Resistor  R=Rd_sw Ohm  enable_R_tol=ee.enum.toleranceApplication.none  R_tol=5  tol_distribution=ee.enum.toleranceDistribution.uniform  nSigma=4  enable_operating_limits=ee.enum.enable.no  operating_limit_action=ee.enum.passive.reportOpLim.warn  power_rating=1 W  max_working_voltage=100 V  noise_mode=ee.enum.sources.noise.Disabled  Tdevice=25 degC  sample_time=1e-3 s  repeatability=ee.enum.ic.repeatability.notRepeatable  user_seed=0  auto_seed=1196140742  power_derating_T1=70 degC  power_derating_T2=155 degC  operating_temperature_range_vec=[-50, 150] degC  alpha=3.93e-3 1/K  Tmeas=25 degC  thermal_mass=100 J/K  temperature_specify=off  temperature_priority=High  temperature=298.15 K  temperature_nominal_specify=off  temperature_nominal_value=1  temperature_nominal_unit=K
  Solver_Configuration : nesl_utility/Solver Configuration  PhysicalDomain=network_engine_domain  SubClassName=solver  LeftPortType=input  RightPortType=generic  Tones=[]  Harmonics=[]  SimulateNoise=off  Profile=off  UseLocalSampling=off  EnableSwitchedLinearOptims=on  FrequencyDomain=off  UseCCode=off  RelTol=0.001  AbsTol=0.001  MinStep=1e-09  ToWorkspace=off  RevertToSquareIcSolve=off  NumHomotopyIterations=100  PhasorMode=off  PhasorModeNumHarmonics=1  ConsistencySolver=NEWTON_XTOL_AFTER_FTOL  IndexReductionMethod=DerivativeReplacement  DoDC=off  ResidualTolerance=1e-09  ConsistencyTolSource=GLOBAL  ConsistencyAbsTol=0.001  ConsistencyRelTol=0.001  ConsistencyTolFactor=0.001  UseLocalSolver=off  LocalSolverChoice=NE_BACKWARD_EULER_ADVANCER  ResolveIndetEquations=on  FunctionEvalNumThread=1  LocalSolverSampleTime=0.001  DoFixedCost=off  MaxNonlinIter=3  MaxModeIter=2  ComputeImpulses=off  ImpulseIterations=2  LinearAlgebra=auto  LinearAlgebraNumThread=0  EquationFormulation=NE_TIME_EF  DelaysMemoryBudget=1024  AutomaticFiltering=on  FilteringTimeConstant=0.001  PartitionStorageMethod=AS_NEEDED  PartitionMemoryBudget=1024  PartitionMethod=ROBUST  MultibodyUseLocalSolver=off  MultibodyLocalSolverChoice=ODE1  MultibodyLocalSolverSampleTime=0.001
  abs_A : Abs  SaturateOnIntegerOverflow=off
  abs_B : Abs  SaturateOnIntegerOverflow=off
  abs_C : Abs  SaturateOnIntegerOverflow=off
  carrier_A : simulink/Sources/Repeating Sequence  rep_seq_t=[0 T_switch/2 T_switch]  rep_seq_y=[0 1 0]
  carrier_B : simulink/Sources/Repeating Sequence  rep_seq_t=[0 T_switch/2 T_switch]  rep_seq_y=[0 1 0]
  carrier_C : simulink/Sources/Repeating Sequence  rep_seq_t=[0 T_switch/2 T_switch]  rep_seq_y=[0 1 0]
  mod_ref_A : Sin  Amplitude=m_index  Frequency=w_grid_sw  SampleTime=0
  mod_ref_B : Sin  Amplitude=m_index  Frequency=w_grid_sw  Phase=-2.0943951023931953  SampleTime=0
  mod_ref_C : Sin  Amplitude=m_index  Frequency=w_grid_sw  Phase=2.0943951023931953  SampleTime=0
  neg_A : Logic  Operator=NOT  AllPortsSameDT=off  OutDataTypeStr=boolean
  neg_B : Logic  Operator=NOT  AllPortsSameDT=off  OutDataTypeStr=boolean
  neg_C : Logic  Operator=NOT  AllPortsSameDT=off  OutDataTypeStr=boolean
  neutral_sign : Gain  Gain=-1
  neutral_sum : Sum  Inputs=+++
  node_CFT_A_024 : ConnectionLabel  Label=CFT_A
  node_CFT_A_025 : ConnectionLabel  Label=CFT_A
  node_CFT_B_046 : ConnectionLabel  Label=CFT_B
  node_CFT_B_047 : ConnectionLabel  Label=CFT_B
  node_CFT_C_068 : ConnectionLabel  Label=CFT_C
  node_CFT_C_069 : ConnectionLabel  Label=CFT_C
  node_C_A_018 : ConnectionLabel  Label=C_A
  node_C_A_019 : ConnectionLabel  Label=C_A
  node_C_A_023 : ConnectionLabel  Label=C_A
  node_C_B_040 : ConnectionLabel  Label=C_B
  node_C_B_041 : ConnectionLabel  Label=C_B
  node_C_B_045 : ConnectionLabel  Label=C_B
  node_C_C_062 : ConnectionLabel  Label=C_C
  node_C_C_063 : ConnectionLabel  Label=C_C
  node_C_C_067 : ConnectionLabel  Label=C_C
  node_GRID_A_022 : ConnectionLabel  Label=GRID_A
  node_GRID_A_027 : ConnectionLabel  Label=GRID_A
  node_GRID_B_044 : ConnectionLabel  Label=GRID_B
  node_GRID_B_049 : ConnectionLabel  Label=GRID_B
  node_GRID_C_066 : ConnectionLabel  Label=GRID_C
  node_GRID_C_071 : ConnectionLabel  Label=GRID_C
  node_I1N_A_016 : ConnectionLabel  Label=I1N_A
  node_I1N_A_017 : ConnectionLabel  Label=I1N_A
  node_I1N_B_038 : ConnectionLabel  Label=I1N_B
  node_I1N_B_039 : ConnectionLabel  Label=I1N_B
  node_I1N_C_060 : ConnectionLabel  Label=I1N_C
  node_I1N_C_061 : ConnectionLabel  Label=I1N_C
  node_L2O_A_020 : ConnectionLabel  Label=L2O_A
  node_L2O_A_021 : ConnectionLabel  Label=L2O_A
  node_L2O_B_042 : ConnectionLabel  Label=L2O_B
  node_L2O_B_043 : ConnectionLabel  Label=L2O_B
  node_L2O_C_064 : ConnectionLabel  Label=L2O_C
  node_L2O_C_065 : ConnectionLabel  Label=L2O_C
  node_M_004 : ConnectionLabel  Label=M
  node_M_010 : ConnectionLabel  Label=M
  node_M_032 : ConnectionLabel  Label=M
  node_M_054 : ConnectionLabel  Label=M
  node_N_002 : ConnectionLabel  Label=N
  node_N_003 : ConnectionLabel  Label=N
  node_N_005 : ConnectionLabel  Label=N
  node_N_006 : ConnectionLabel  Label=N
  node_N_011 : ConnectionLabel  Label=N
  node_N_026 : ConnectionLabel  Label=N
  node_N_028 : ConnectionLabel  Label=N
  node_N_033 : ConnectionLabel  Label=N
  node_N_048 : ConnectionLabel  Label=N
  node_N_050 : ConnectionLabel  Label=N
  node_N_055 : ConnectionLabel  Label=N
  node_N_070 : ConnectionLabel  Label=N
  node_N_072 : ConnectionLabel  Label=N
  node_P_001 : ConnectionLabel  Label=P
  node_P_007 : ConnectionLabel  Label=P
  node_P_029 : ConnectionLabel  Label=P
  node_P_051 : ConnectionLabel  Label=P
  node_X_A_008 : ConnectionLabel  Label=X_A
  node_X_A_009 : ConnectionLabel  Label=X_A
  node_X_A_013 : ConnectionLabel  Label=X_A
  node_X_A_015 : ConnectionLabel  Label=X_A
  node_X_B_030 : ConnectionLabel  Label=X_B
  node_X_B_031 : ConnectionLabel  Label=X_B
  node_X_B_035 : ConnectionLabel  Label=X_B
  node_X_B_037 : ConnectionLabel  Label=X_B
  node_X_C_052 : ConnectionLabel  Label=X_C
  node_X_C_053 : ConnectionLabel  Label=X_C
  node_X_C_057 : ConnectionLabel  Label=X_C
  node_X_C_059 : ConnectionLabel  Label=X_C
  node_Z_A_012 : ConnectionLabel  Label=Z_A
  node_Z_A_014 : ConnectionLabel  Label=Z_A
  node_Z_B_034 : ConnectionLabel  Label=Z_B
  node_Z_B_036 : ConnectionLabel  Label=Z_B
  node_Z_C_056 : ConnectionLabel  Label=Z_C
  node_Z_C_058 : ConnectionLabel  Label=Z_C
  not_pwm_A : Logic  Operator=NOT  AllPortsSameDT=off  OutDataTypeStr=boolean
  not_pwm_B : Logic  Operator=NOT  AllPortsSameDT=off  OutDataTypeStr=boolean
  not_pwm_C : Logic  Operator=NOT  AllPortsSameDT=off  OutDataTypeStr=boolean
  pos_A : RelationalOperator  OutDataTypeStr=boolean  RndMeth=Simplest  InputSameDT=off
  pos_B : RelationalOperator  OutDataTypeStr=boolean  RndMeth=Simplest  InputSameDT=off
  pos_C : RelationalOperator  OutDataTypeStr=boolean  RndMeth=Simplest  InputSameDT=off
  pwm_A : RelationalOperator  OutDataTypeStr=boolean  RndMeth=Simplest  InputSameDT=off
  pwm_B : RelationalOperator  OutDataTypeStr=boolean  RndMeth=Simplest  InputSameDT=off
  pwm_C : RelationalOperator  OutDataTypeStr=boolean  RndMeth=Simplest  InputSameDT=off
  save_A_Q1 : ToWorkspace  VariableName=a_q1_3sw_log  SaveFormat=Timeseries  SampleTime=-1
  save_A_Q2 : ToWorkspace  VariableName=a_q2_3sw_log  SaveFormat=Timeseries  SampleTime=-1
  save_A_Q3 : ToWorkspace  VariableName=a_q3_3sw_log  SaveFormat=Timeseries  SampleTime=-1
  save_A_Q4 : ToWorkspace  VariableName=a_q4_3sw_log  SaveFormat=Timeseries  SampleTime=-1
  save_B_Q1 : ToWorkspace  VariableName=b_q1_3sw_log  SaveFormat=Timeseries  SampleTime=-1
  save_B_Q2 : ToWorkspace  VariableName=b_q2_3sw_log  SaveFormat=Timeseries  SampleTime=-1
  save_B_Q3 : ToWorkspace  VariableName=b_q3_3sw_log  SaveFormat=Timeseries  SampleTime=-1
  save_B_Q4 : ToWorkspace  VariableName=b_q4_3sw_log  SaveFormat=Timeseries  SampleTime=-1
  save_C_Q1 : ToWorkspace  VariableName=c_q1_3sw_log  SaveFormat=Timeseries  SampleTime=-1
  save_C_Q2 : ToWorkspace  VariableName=c_q2_3sw_log  SaveFormat=Timeseries  SampleTime=-1
  save_C_Q3 : ToWorkspace  VariableName=c_q3_3sw_log  SaveFormat=Timeseries  SampleTime=-1
  save_C_Q4 : ToWorkspace  VariableName=c_q4_3sw_log  SaveFormat=Timeseries  SampleTime=-1
  save_I1_A : ToWorkspace  VariableName=i1_a_3sw_log  SaveFormat=Timeseries  SampleTime=-1
  save_I1_B : ToWorkspace  VariableName=i1_b_3sw_log  SaveFormat=Timeseries  SampleTime=-1
  save_I1_C : ToWorkspace  VariableName=i1_c_3sw_log  SaveFormat=Timeseries  SampleTime=-1
  save_Ig_A : ToWorkspace  VariableName=ig_a_3sw_log  SaveFormat=Timeseries  SampleTime=-1
  save_Ig_B : ToWorkspace  VariableName=ig_b_3sw_log  SaveFormat=Timeseries  SampleTime=-1
  save_Ig_C : ToWorkspace  VariableName=ig_c_3sw_log  SaveFormat=Timeseries  SampleTime=-1
  save_neutral : ToWorkspace  VariableName=i_neutral_3sw_log  SaveFormat=Timeseries  SampleTime=-1
  zero_A : Constant  Value=0
  zero_B : Constant  Value=0
  zero_C : Constant  Value=0
  wires:
  mod_ref_A/1 -> abs_A/1, pos_A/1
  abs_A/1 -> pwm_A/1
  carrier_A/1 -> pwm_A/2
  zero_A/1 -> pos_A/2
  pos_A/1 -> neg_A/1, A_Q1_gate/1, A_Q3_gate/1
  pwm_A/1 -> not_pwm_A/1, A_Q1_gate/2, A_Q2_gate/2
  neg_A/1 -> A_Q2_gate/1, A_Q4_gate/1
  not_pwm_A/1 -> A_Q3_gate/2, A_Q4_gate/2
  A_Q1_gate/1 -> A_Q1_double/1
  A_Q1_double/1 -> A_Q1_delay/1, A_Q1_actual/1
  A_Q1_delay/1 -> A_Q1_actual/2
  A_Q1_actual/1 -> A_Q1_PS/1, save_A_Q1/1
  A_Q2_gate/1 -> A_Q2_double/1
  A_Q2_double/1 -> A_Q2_delay/1, A_Q2_actual/1
  A_Q2_delay/1 -> A_Q2_actual/2
  A_Q2_actual/1 -> A_Q2_PS/1, save_A_Q2/1
  A_Q3_gate/1 -> A_Q3_double/1
  A_Q3_double/1 -> A_Q3_delay/1, A_Q3_actual/1
  A_Q3_delay/1 -> A_Q3_actual/2
  A_Q3_actual/1 -> A_Q3_PS/1, save_A_Q3/1
  A_Q4_gate/1 -> A_Q4_double/1
  A_Q4_double/1 -> A_Q4_delay/1, A_Q4_actual/1
  A_Q4_delay/1 -> A_Q4_actual/2
  A_Q4_actual/1 -> A_Q4_PS/1, save_A_Q4/1
  I1_PS_A/1 -> save_I1_A/1
  Ig_PS_A/1 -> save_Ig_A/1, neutral_sum/1
  mod_ref_B/1 -> abs_B/1, pos_B/1
  abs_B/1 -> pwm_B/1
  carrier_B/1 -> pwm_B/2
  zero_B/1 -> pos_B/2
  pos_B/1 -> neg_B/1, B_Q1_gate/1, B_Q3_gate/1
  pwm_B/1 -> not_pwm_B/1, B_Q1_gate/2, B_Q2_gate/2
  neg_B/1 -> B_Q2_gate/1, B_Q4_gate/1
  not_pwm_B/1 -> B_Q3_gate/2, B_Q4_gate/2
  B_Q1_gate/1 -> B_Q1_double/1
  B_Q1_double/1 -> B_Q1_delay/1, B_Q1_actual/1
  B_Q1_delay/1 -> B_Q1_actual/2
  B_Q1_actual/1 -> B_Q1_PS/1, save_B_Q1/1
  B_Q2_gate/1 -> B_Q2_double/1
  B_Q2_double/1 -> B_Q2_delay/1, B_Q2_actual/1
  B_Q2_delay/1 -> B_Q2_actual/2
  B_Q2_actual/1 -> B_Q2_PS/1, save_B_Q2/1
  B_Q3_gate/1 -> B_Q3_double/1
  B_Q3_double/1 -> B_Q3_delay/1, B_Q3_actual/1
  B_Q3_delay/1 -> B_Q3_actual/2
  B_Q3_actual/1 -> B_Q3_PS/1, save_B_Q3/1
  B_Q4_gate/1 -> B_Q4_double/1
  B_Q4_double/1 -> B_Q4_delay/1, B_Q4_actual/1
  B_Q4_delay/1 -> B_Q4_actual/2
  B_Q4_actual/1 -> B_Q4_PS/1, save_B_Q4/1
  I1_PS_B/1 -> save_I1_B/1
  Ig_PS_B/1 -> save_Ig_B/1, neutral_sum/2
  mod_ref_C/1 -> abs_C/1, pos_C/1
  abs_C/1 -> pwm_C/1
  carrier_C/1 -> pwm_C/2
  zero_C/1 -> pos_C/2
  pos_C/1 -> neg_C/1, C_Q1_gate/1, C_Q3_gate/1
  pwm_C/1 -> not_pwm_C/1, C_Q1_gate/2, C_Q2_gate/2
  neg_C/1 -> C_Q2_gate/1, C_Q4_gate/1
  not_pwm_C/1 -> C_Q3_gate/2, C_Q4_gate/2
  C_Q1_gate/1 -> C_Q1_double/1
  C_Q1_double/1 -> C_Q1_delay/1, C_Q1_actual/1
  C_Q1_delay/1 -> C_Q1_actual/2
  C_Q1_actual/1 -> C_Q1_PS/1, save_C_Q1/1
  C_Q2_gate/1 -> C_Q2_double/1
  C_Q2_double/1 -> C_Q2_delay/1, C_Q2_actual/1
  C_Q2_delay/1 -> C_Q2_actual/2
  C_Q2_actual/1 -> C_Q2_PS/1, save_C_Q2/1
  C_Q3_gate/1 -> C_Q3_double/1
  C_Q3_double/1 -> C_Q3_delay/1, C_Q3_actual/1
  C_Q3_delay/1 -> C_Q3_actual/2
  C_Q3_actual/1 -> C_Q3_PS/1, save_C_Q3/1
  C_Q4_gate/1 -> C_Q4_double/1
  C_Q4_double/1 -> C_Q4_delay/1, C_Q4_actual/1
  C_Q4_delay/1 -> C_Q4_actual/2
  C_Q4_actual/1 -> C_Q4_PS/1, save_C_Q4/1
  I1_PS_C/1 -> save_I1_C/1
  Ig_PS_C/1 -> save_Ig_C/1, neutral_sum/3
  neutral_sum/1 -> neutral_sign/1
  neutral_sign/1 -> save_neutral/1
  connections:
  DC_top/LConn1 -- node_P_001/LConn1
  DC_top/RConn1 -- node_N_002/LConn1
  DC_bottom/LConn1 -- node_N_003/LConn1
  DC_bottom/RConn1 -- node_M_004/LConn1
  Electrical_reference/LConn1 -- node_N_005/LConn1
  Solver_Configuration/RConn1 -- node_N_006/LConn1
  A_Q1_PS/RConn1 -- A_Q1/LConn1
  A_Q2_PS/RConn1 -- A_Q2/LConn1
  A_Q3_PS/RConn1 -- A_Q3/LConn1
  A_Q4_PS/RConn1 -- A_Q4/LConn1
  A_Q1/RConn1 -- node_P_007/LConn1
  A_Q1/RConn2 -- node_X_A_008/LConn1
  A_Q2/RConn1 -- node_X_A_009/LConn1
  A_Q2/RConn2 -- node_M_010/LConn1
  A_Q3/RConn1 -- node_N_011/LConn1
  A_Q3/RConn2 -- node_Z_A_012/LConn1
  A_Q4/RConn1 -- node_X_A_013/LConn1
  A_Q4/RConn2 -- node_Z_A_014/LConn1
  I1_sensor_A/LConn1 -- node_X_A_015/LConn1
  I1_sensor_A/RConn2 -- node_I1N_A_016/LConn1
  L1_A/LConn1 -- node_I1N_A_017/LConn1
  L1_A/RConn1 -- node_C_A_018/LConn1
  L2_A/LConn1 -- node_C_A_019/LConn1
  L2_A/RConn1 -- node_L2O_A_020/LConn1
  Grid_sensor_A/LConn1 -- node_L2O_A_021/LConn1
  Grid_sensor_A/RConn2 -- node_GRID_A_022/LConn1
  Rd_A/LConn1 -- node_C_A_023/LConn1
  Rd_A/RConn1 -- node_CFT_A_024/LConn1
  Cf_A/LConn1 -- node_CFT_A_025/LConn1
  Cf_A/RConn1 -- node_N_026/LConn1
  Grid_source_A/LConn1 -- node_GRID_A_027/LConn1
  Grid_source_A/RConn1 -- node_N_028/LConn1
  I1_sensor_A/RConn1 -- I1_PS_A/LConn1
  Grid_sensor_A/RConn1 -- Ig_PS_A/LConn1
  B_Q1_PS/RConn1 -- B_Q1/LConn1
  B_Q2_PS/RConn1 -- B_Q2/LConn1
  B_Q3_PS/RConn1 -- B_Q3/LConn1
  B_Q4_PS/RConn1 -- B_Q4/LConn1
  B_Q1/RConn1 -- node_P_029/LConn1
  B_Q1/RConn2 -- node_X_B_030/LConn1
  B_Q2/RConn1 -- node_X_B_031/LConn1
  B_Q2/RConn2 -- node_M_032/LConn1
  B_Q3/RConn1 -- node_N_033/LConn1
  B_Q3/RConn2 -- node_Z_B_034/LConn1
  B_Q4/RConn1 -- node_X_B_035/LConn1
  B_Q4/RConn2 -- node_Z_B_036/LConn1
  I1_sensor_B/LConn1 -- node_X_B_037/LConn1
  I1_sensor_B/RConn2 -- node_I1N_B_038/LConn1
  L1_B/LConn1 -- node_I1N_B_039/LConn1
  L1_B/RConn1 -- node_C_B_040/LConn1
  L2_B/LConn1 -- node_C_B_041/LConn1
  L2_B/RConn1 -- node_L2O_B_042/LConn1
  Grid_sensor_B/LConn1 -- node_L2O_B_043/LConn1
  Grid_sensor_B/RConn2 -- node_GRID_B_044/LConn1
  Rd_B/LConn1 -- node_C_B_045/LConn1
  Rd_B/RConn1 -- node_CFT_B_046/LConn1
  Cf_B/LConn1 -- node_CFT_B_047/LConn1
  Cf_B/RConn1 -- node_N_048/LConn1
  Grid_source_B/LConn1 -- node_GRID_B_049/LConn1
  Grid_source_B/RConn1 -- node_N_050/LConn1
  I1_sensor_B/RConn1 -- I1_PS_B/LConn1
  Grid_sensor_B/RConn1 -- Ig_PS_B/LConn1
  C_Q1_PS/RConn1 -- C_Q1/LConn1
  C_Q2_PS/RConn1 -- C_Q2/LConn1
  C_Q3_PS/RConn1 -- C_Q3/LConn1
  C_Q4_PS/RConn1 -- C_Q4/LConn1
  C_Q1/RConn1 -- node_P_051/LConn1
  C_Q1/RConn2 -- node_X_C_052/LConn1
  C_Q2/RConn1 -- node_X_C_053/LConn1
  C_Q2/RConn2 -- node_M_054/LConn1
  C_Q3/RConn1 -- node_N_055/LConn1
  C_Q3/RConn2 -- node_Z_C_056/LConn1
  C_Q4/RConn1 -- node_X_C_057/LConn1
  C_Q4/RConn2 -- node_Z_C_058/LConn1
  I1_sensor_C/LConn1 -- node_X_C_059/LConn1
  I1_sensor_C/RConn2 -- node_I1N_C_060/LConn1
  L1_C/LConn1 -- node_I1N_C_061/LConn1
  L1_C/RConn1 -- node_C_C_062/LConn1
  L2_C/LConn1 -- node_C_C_063/LConn1
  L2_C/RConn1 -- node_L2O_C_064/LConn1
  Grid_sensor_C/LConn1 -- node_L2O_C_065/LConn1
  Grid_sensor_C/RConn2 -- node_GRID_C_066/LConn1
  Rd_C/LConn1 -- node_C_C_067/LConn1
  Rd_C/RConn1 -- node_CFT_C_068/LConn1
  Cf_C/LConn1 -- node_CFT_C_069/LConn1
  Cf_C/RConn1 -- node_N_070/LConn1
  Grid_source_C/LConn1 -- node_GRID_C_071/LConn1
  Grid_source_C/RConn1 -- node_N_072/LConn1
  I1_sensor_C/RConn1 -- I1_PS_C/LConn1
  Grid_sensor_C/RConn1 -- Ig_PS_C/LConn1
